simulink library "QD2_Mission_Lib"  (R2022b)
settings: Solver=VariableStepAuto  StartTime=0.0  StopTime=10.0  RelTol=1e-3
undefined symbols (not defined in the file): QD2P
settings Model: Creator=ezequ  LastModifiedBy=ezequ
settings OptimizationCC: ReuseModelBlockBuffer=on
settings RTWCC: GPUComputeCapability=5.0
settings ConfigComp: CovBoundaryAbsTol=1.0e-5

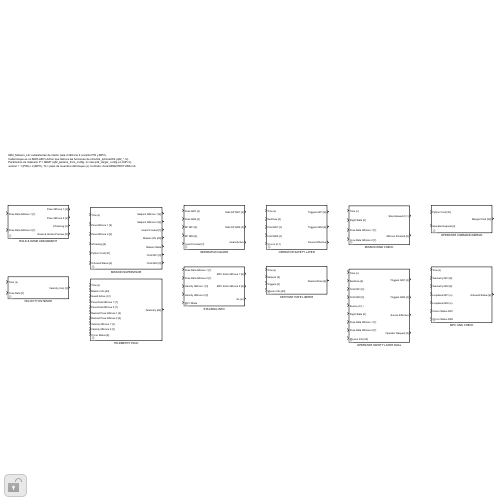
[thumbnail: Simulink's stored preview of the top-level diagram]
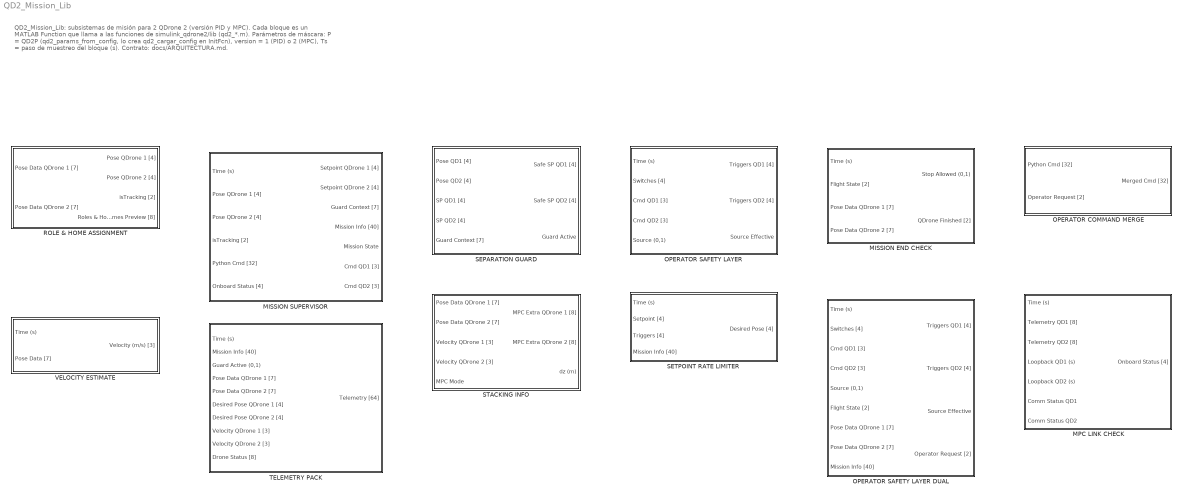
== system QD2_Mission_Lib ==
  note: QD2_Mission_Lib: subsistemas de misión para 2 QDrone 2 (versión PID y MPC).
      | Cada bloque es un MATLAB Function que llama a las funciones de simulink_qdrone2/lib (qd2_*.m).
      | Parámetros de máscara: P = QD2P (qd2_params_from_config, lo crea qd2_cargar_config en InitFcn),
      | version = 1 (PID) o 2 (MPC), Ts = paso de muestreo del bloque (s). Contrato: docs/ARQUITECTURA.md.
  MISSION END CHECK : Subsystem  TreatAsAtomicUnit=on  SystemSampleTime=Ts  mask(QD2 Mission Lib){Ts=0.001}
      mask prompts: Ts "Paso de muestreo (s):"
      mask help: CORRECCIÓN del paro automático del original (paraba 3 s después de Land aunque el dron siguiera en el aire). Un dron "terminó" si su Flight_State es 3 (Land) o 9 (MS Stop) Y está en el suelo (rastreado, z < 0.10 m) durante 3 s seguidos, o lleva 60 s SEGUIDOS sin rastreo en 3/9 (respaldo). Un dron rastreado con z >= 0.10 m NUNCA permite el paro. Stop Allowed = los dos terminaron (o nunca se armaron) y al menos uno se armó. El Stop with Message del Flight Plan solo actúa con Stop Allowed = 1.
  MISSION SUPERVISOR : Subsystem  TreatAsAtomicUnit=on  SystemSampleTime=Ts  mask(QD2 Mission Lib){P=QD2P, version=1, Ts=0.001}
      mask prompts: P "Parámetros de misión (struct de qd2_params_from_config):"; version "Versión (1 = PID, 2 = MPC):"; Ts "Paso de muestreo (s):"
      mask help: FSM de misión (qd2_mission_step, ARQUITECTURA §3.3). Commands = [arm takeoff estop] por dron: el OPERATOR SAFETY LAYER los combina con los switches del operador. Guard Context = [explorer_id ctx_guard(6)]. Onboard Status [4] = [fsm1 fsm2 cod1 cod2] del MPC LINK CHECK (versión MPC; en PID constante 0 = desconocido; cod 1 = protocolo MPC incorrecto, 2 = enlace perdido): un dron en vuelo con FSM a bordo 7/8/9 o sin enlace (o protocolo incorrecto) -> alerta 9 (10), el sano se aparta >= d_min_h a su altura, regresa y aterriza; DONE. En LANDING, R no baja hasta que E está a >= d_min_h en horizontal. Mission Info [40] = campos de telemetría para el TELEMETRY PACK (ver codigo_supervisor en construir_modelos.m).
  MPC LINK CHECK : Subsystem  TreatAsAtomicUnit=on  SystemSampleTime=Ts  mask(QD2 Mission Lib){P=QD2P, version=1, Ts=0.001}
      mask prompts: P "Parámetros de misión (struct de qd2_params_from_config):"; version "Versión (1 = PID, 2 = MPC):"; Ts "Paso de muestreo (s):"
      mask help: Versión MPC (qd2_enlace_mpc): valida la respuesta de 8 doubles de cada dron (§3.2): válida si y(8) = 2 (etiqueta protocolo MPC v1) y la FSM y(2) es un entero 1..9. Si el dron está conectado (loopback < 0.5 s y sin pérdida de enlace) y responde mal más de 0.5 s seguidos -> protocolo incorrecto (cod 1, alerta 10, dron no disponible). Sin conexión después de haber estado conectado -> enlace perdido (cod 2; la FSM retenida no se usa: fsm = 0). Onboard Status = [fsm1 fsm2 cod1 cod2] (fsm 0 = desconocida) -> MISSION SUPERVISOR. Con version = 1 (PID, el dron solo devuelve el eco) la salida es 0.
  OPERATOR COMMAND MERGE : Subsystem  TreatAsAtomicUnit=on  SystemSampleTime=Ts  mask(QD2 Mission Lib){Ts=0.001}
      mask prompts: Ts "Paso de muestreo (s):"
      mask help: Inyecta LAND ALL (cmd 3) en el flujo de comandos de Python cuando el OPERATOR SAFETY LAYER DUAL lo pide (contador Operator Request(1) cambia). Paso 1: heartbeat y cmd_seq distintos -> el supervisor lo acepta aunque la estación Python esté caída. Paso 2: vuelve a la secuencia real de Python SIN comando, así el último comando de Python no se re-ejecuta. La entrada Operator Request debe llegar con 1 paso de retardo.
  OPERATOR SAFETY LAYER : Subsystem  TreatAsAtomicUnit=on  SystemSampleTime=Ts  mask(QD2 Mission Lib){Ts=0.001}
      mask prompts: Ts "Paso de muestreo (s):"
      mask help: Versión SIMPLE (la usa QD2_Sim_Dual; interfaz de 5/3 puertos sin cambios). Los modelos de tierra usan OPERATOR SAFETY LAYER DUAL. En modo MISIÓN (Command Source = 0) arm_i = switch AND misión, takeoff_i = switch AND misión (solo tras >= 1 s armado), estop_i = switch OR misión. En modo MANUAL Equipo2 (1) el dron 1 recibe los switches (takeoff también >= 1 s después de armar) y el dron 2 solo el E-stop. El modo solo cambia con los dos drones desarmados Y los switches Arm y Takeoff abajo (nunca se dispara solo).
  OPERATOR SAFETY LAYER DUAL : Subsystem  TreatAsAtomicUnit=on  SystemSampleTime=Ts  mask(QD2 Mission Lib){P=QD2P, Ts=0.001}
      mask prompts: P "Parámetros de misión (struct de qd2_params_from_config):"; Ts "Paso de muestreo (s):"
      mask help: Capa de seguridad del operador (modelos de tierra). Switches = autoridad final. MISIÓN: arm_i = switch AND misión; Takeoff/Land arriba = PERMISO de despegue (takeoff >= 1 s después de armar); en vuelo, BAJARLO pide LAND ALL al supervisor (Operator Request -> OPERATOR COMMAND MERGE): aterrizaje ordenado, R primero y E se aparta; el takeoff de cada dron sigue al supervisor. Respaldo crudo si el supervisor no acepta en 2 s o tras 90 s: suelta el takeoff, pero NUNCA el de un dron que tiene al otro debajo a < d_min_h. E-stop = corte inmediato. Arm abajo / E-stop en vuelo también piden LAND ALL. MANUAL: como el original (solo dron 1) con takeoff >= 1 s después de armar. El modo solo cambia en tierra: Flight State [0 0], desarmados, switches Arm y Takeoff abajo. Operator Request = [contador de peticiones, alerta 5 E-stop / 6 Takeoff abajo / 7 Arm abajo / 8 respaldo crudo].
  ROLE & HOME ASSIGNMENT : Subsystem  TreatAsAtomicUnit=on  SystemSampleTime=Ts  mask(QD2 Mission Lib){P=QD2P, version=1, Ts=0.001}
      mask prompts: P "Parámetros de misión (struct de qd2_params_from_config):"; version "Versión (1 = PID, 2 = MPC):"; Ts "Paso de muestreo (s):"
      mask help: Separa [x y z yaw] e isTracking de cada dron (Corrected Pose Data [7] = [x y z roll pitch yaw isTracking]) y muestra en vivo la asignación de roles de qd2_assign_roles: [explorer_id responder_id home1(2) home2(2) d_homes start_ok]. El dron con menor x es el EXPLORADOR. El MISSION SUPERVISOR fija roles y homes al recibir START; start_ok = 0 avisa ANTES de START que los homes están demasiado cerca (START se rechazaría, alerta 1).
  SEPARATION GUARD : Subsystem  TreatAsAtomicUnit=on  SystemSampleTime=Ts  mask(QD2 Mission Lib){P=QD2P, Ts=0.001}
      mask prompts: P "Parámetros de misión (struct de qd2_params_from_config):"; Ts "Paso de muestreo (s):"
      mask help: Versión PID: nunca uno encima del otro (qd2_separation_guard). Distancia horizontal >= d_min_h entre poses, consignas y caminos rectos. Traduce dron <-> rol con explorer_id (Guard Context(1)) y reinicia su estado si los roles cambian. Después de este bloque la consigna DEBE limitarse por norma (SETPOINT RATE LIMITER).
  SETPOINT RATE LIMITER : Subsystem  TreatAsAtomicUnit=on  SystemSampleTime=Ts  mask(QD2 Mission Lib){P=QD2P, dron=1, Ts=0.001}
      mask prompts: P "Parámetros de misión (struct de qd2_params_from_config):"; dron "QDrone (1 o 2):"; Ts "Paso de muestreo (s):"
      mask help: Saturation (como Saturation2 original, con z hasta P.z_max) + limitador de razón por NORMA en x,y (qd2_rate_limit(...,1)): 1/3 m/s xy, 1/6 m/s z, 30 °/s yaw. Sustituye al Rate Limiter2 por eje (que hace caminos en L y rompe la separación). Desarmado (Triggers(1) = 0) la consigna pasa sin limitar. Mientras este dron se aparta de un dron en falla a bordo (Mission Info(37 + dron) = 1) el límite xy es P.falla_rate_xy (1 m/s). Parámetro dron = 1 o 2.
  STACKING INFO : Subsystem  TreatAsAtomicUnit=on  SystemSampleTime=Ts  mask(QD2 Mission Lib){Ts=0.001}
      mask prompts: Ts "Paso de muestreo (s):"
      mask help: Versión MPC: índices 17-24 del mensaje de 24 doubles (§3.2) para cada dron = [x y z vx vy vz del OTRO dron, mpc_mode, 2]. El índice 24 = 2 es la etiqueta "protocolo MPC v1": el PROTOCOL CHECK a bordo solo acepta tramas con 24 = 2. Si el otro no está rastreado se mandan NaN (el MPC a bordo desactiva el feedforward de downwash).
  TELEMETRY PACK : Subsystem  TreatAsAtomicUnit=on  SystemSampleTime=Ts  mask(QD2 Mission Lib){version=1, Ts=0.001}
      mask prompts: version "Versión (1 = PID, 2 = MPC):"; Ts "Paso de muestreo (s):"
      mask help: Arma los 64 doubles Simulink -> Python (§3.3) con qd2_telemetry_pack. Drone Status = [fsm1 fsm2 bat1 bat2 comm_issue1 comm_issue2 loopback1 loopback2 (n_peticiones alerta_operador)]; comm_ok = sin issue y loopback < 0.5 s. y(55) = alerta: la del operador (5-8) si hay, si no la del supervisor (0-4, 9 falla a bordo, 10 protocolo MPC incorrecto). y(56:60) = un objetivo por mensaje, rotando: [id clase x y estado]. y(61:63) = [roll pitch válido] del EXPLORADOR (rad), de Pose Data(4:5) del mismo dron (OptiTrack, R = Rz(yaw)Ry(pitch)Rx(roll)); 0 0 0 sin explorador, sin rastreo o con ángulos no finitos. y(64) = 0.
  VELOCITY ESTIMATE : Subsystem  TreatAsAtomicUnit=on  SystemSampleTime=Ts  mask(QD2 Mission Lib){Ts=0.001}
      mask prompts: Ts "Paso de muestreo (s):"
      mask help: Velocidad [vx vy vz] a partir de OptiTrack: derivada entre muestras nuevas (100 Hz) + filtro de primer orden (tau = 0.04 s). Sin rastreo -> 0.

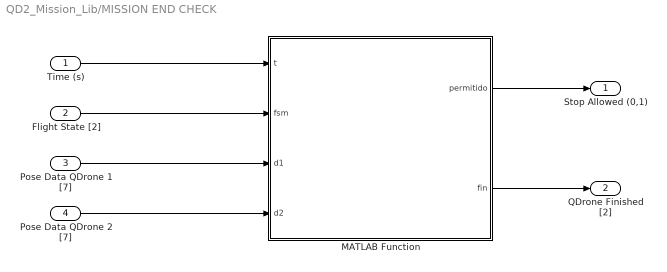
== system QD2_Mission_Lib/MISSION END CHECK ==
  Time (s) : Inport
  Flight State [2] : Inport  Port=2
  Pose Data QDrone 1 [7] : Inport  Port=3
  Pose Data QDrone 2 [7] : Inport  Port=4
  MATLAB Function : MATLAB Function  TreatAsAtomicUnit=on
  Stop Allowed (0,1) : Outport
  QDrone Finished [2] : Outport  Port=2
  wires:
  Time (s)/1 -> MATLAB Function/1(t)
  Flight State [2]/1 -> MATLAB Function/2(fsm)
  Pose Data QDrone 1 [7]/1 -> MATLAB Function/3(d1)
  Pose Data QDrone 2 [7]/1 -> MATLAB Function/4(d2)
  MATLAB Function/1(permitido) -> Stop Allowed (0,1)/1
  MATLAB Function/2(fin) -> QDrone Finished [2]/1

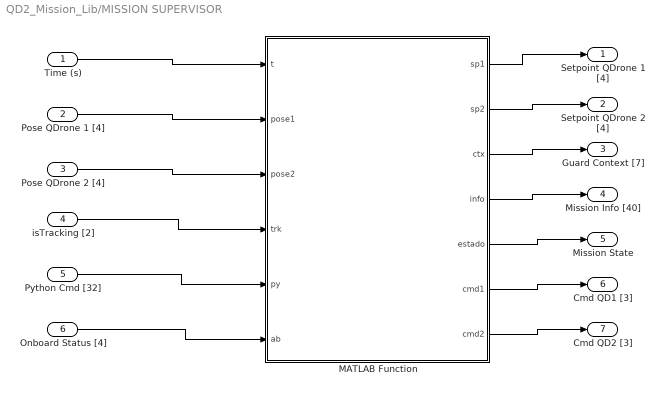
== system QD2_Mission_Lib/MISSION SUPERVISOR ==
  Time (s) : Inport
  Pose QDrone 1 [4] : Inport  Port=2
  Pose QDrone 2 [4] : Inport  Port=3
  isTracking [2] : Inport  Port=4
  Python Cmd [32] : Inport  Port=5
  Onboard Status [4] : Inport  Port=6
  MATLAB Function : MATLAB Function  TreatAsAtomicUnit=on
  Setpoint QDrone 1 [4] : Outport
  Setpoint QDrone 2 [4] : Outport  Port=2
  Guard Context [7] : Outport  Port=3
  Mission Info [40] : Outport  Port=4
  Mission State : Outport  Port=5
  Cmd QD1 [3] : Outport  Port=6
  Cmd QD2 [3] : Outport  Port=7
  wires:
  Time (s)/1 -> MATLAB Function/1(t)
  Pose QDrone 1 [4]/1 -> MATLAB Function/2(pose1)
  Pose QDrone 2 [4]/1 -> MATLAB Function/3(pose2)
  isTracking [2]/1 -> MATLAB Function/4(trk)
  Python Cmd [32]/1 -> MATLAB Function/5(py)
  Onboard Status [4]/1 -> MATLAB Function/6(ab)
  MATLAB Function/1(sp1) -> Setpoint QDrone 1 [4]/1
  MATLAB Function/2(sp2) -> Setpoint QDrone 2 [4]/1
  MATLAB Function/3(ctx) -> Guard Context [7]/1
  MATLAB Function/4(info) -> Mission Info [40]/1
  MATLAB Function/5(estado) -> Mission State/1
  MATLAB Function/6(cmd1) -> Cmd QD1 [3]/1
  MATLAB Function/7(cmd2) -> Cmd QD2 [3]/1

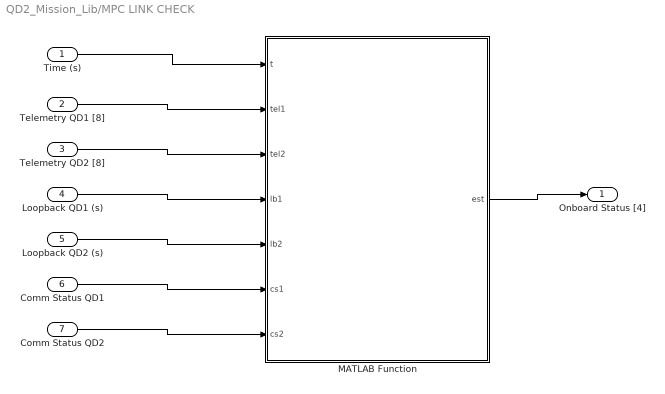
== system QD2_Mission_Lib/MPC LINK CHECK ==
  Time (s) : Inport
  Telemetry QD1 [8] : Inport  Port=2
  Telemetry QD2 [8] : Inport  Port=3
  Loopback QD1 (s) : Inport  Port=4
  Loopback QD2 (s) : Inport  Port=5
  Comm Status QD1 : Inport  Port=6
  Comm Status QD2 : Inport  Port=7
  MATLAB Function : MATLAB Function  TreatAsAtomicUnit=on
  Onboard Status [4] : Outport
  wires:
  Time (s)/1 -> MATLAB Function/1(t)
  Telemetry QD1 [8]/1 -> MATLAB Function/2(tel1)
  Telemetry QD2 [8]/1 -> MATLAB Function/3(tel2)
  Loopback QD1 (s)/1 -> MATLAB Function/4(lb1)
  Loopback QD2 (s)/1 -> MATLAB Function/5(lb2)
  Comm Status QD1/1 -> MATLAB Function/6(cs1)
  Comm Status QD2/1 -> MATLAB Function/7(cs2)
  MATLAB Function/1(est) -> Onboard Status [4]/1

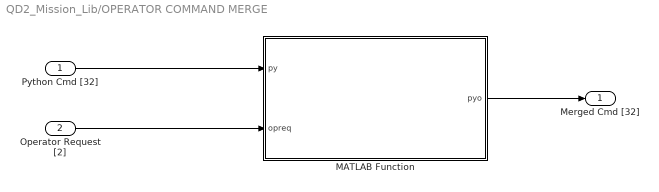
== system QD2_Mission_Lib/OPERATOR COMMAND MERGE ==
  Python Cmd [32] : Inport
  Operator Request [2] : Inport  Port=2
  MATLAB Function : MATLAB Function  TreatAsAtomicUnit=on
  Merged Cmd [32] : Outport
  wires:
  Python Cmd [32]/1 -> MATLAB Function/1(py)
  Operator Request [2]/1 -> MATLAB Function/2(opreq)
  MATLAB Function/1(pyo) -> Merged Cmd [32]/1

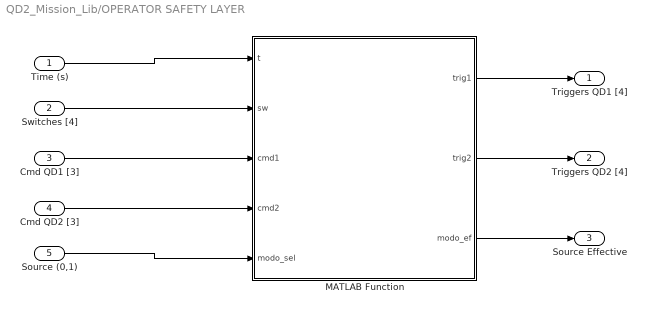
== system QD2_Mission_Lib/OPERATOR SAFETY LAYER ==
  Time (s) : Inport
  Switches [4] : Inport  Port=2
  Cmd QD1 [3] : Inport  Port=3
  Cmd QD2 [3] : Inport  Port=4
  Source (0,1) : Inport  Port=5
  MATLAB Function : MATLAB Function  TreatAsAtomicUnit=on
  Triggers QD1 [4] : Outport
  Triggers QD2 [4] : Outport  Port=2
  Source Effective : Outport  Port=3
  wires:
  Time (s)/1 -> MATLAB Function/1(t)
  Switches [4]/1 -> MATLAB Function/2(sw)
  Cmd QD1 [3]/1 -> MATLAB Function/3(cmd1)
  Cmd QD2 [3]/1 -> MATLAB Function/4(cmd2)
  Source (0,1)/1 -> MATLAB Function/5(modo_sel)
  MATLAB Function/1(trig1) -> Triggers QD1 [4]/1
  MATLAB Function/2(trig2) -> Triggers QD2 [4]/1
  MATLAB Function/3(modo_ef) -> Source Effective/1

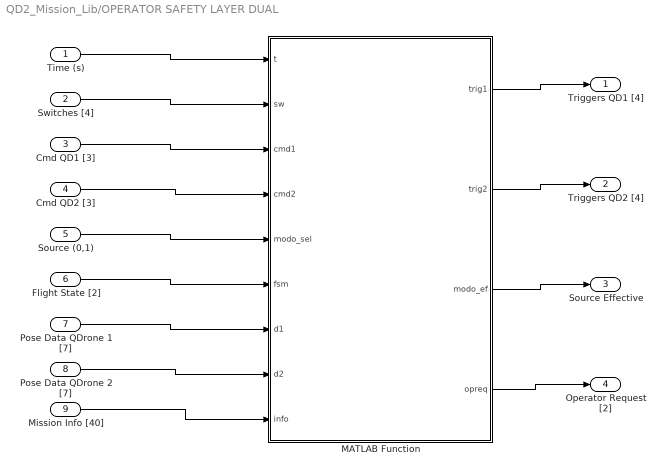
== system QD2_Mission_Lib/OPERATOR SAFETY LAYER DUAL ==
  Time (s) : Inport
  Switches [4] : Inport  Port=2
  Cmd QD1 [3] : Inport  Port=3
  Cmd QD2 [3] : Inport  Port=4
  Source (0,1) : Inport  Port=5
  Flight State [2] : Inport  Port=6
  Pose Data QDrone 1 [7] : Inport  Port=7
  Pose Data QDrone 2 [7] : Inport  Port=8
  Mission Info [40] : Inport  Port=9
  MATLAB Function : MATLAB Function  TreatAsAtomicUnit=on
  Triggers QD1 [4] : Outport
  Triggers QD2 [4] : Outport  Port=2
  Source Effective : Outport  Port=3
  Operator Request [2] : Outport  Port=4
  wires:
  Time (s)/1 -> MATLAB Function/1(t)
  Switches [4]/1 -> MATLAB Function/2(sw)
  Cmd QD1 [3]/1 -> MATLAB Function/3(cmd1)
  Cmd QD2 [3]/1 -> MATLAB Function/4(cmd2)
  Source (0,1)/1 -> MATLAB Function/5(modo_sel)
  Flight State [2]/1 -> MATLAB Function/6(fsm)
  Pose Data QDrone 1 [7]/1 -> MATLAB Function/7(d1)
  Pose Data QDrone 2 [7]/1 -> MATLAB Function/8(d2)
  Mission Info [40]/1 -> MATLAB Function/9(info)
  MATLAB Function/1(trig1) -> Triggers QD1 [4]/1
  MATLAB Function/2(trig2) -> Triggers QD2 [4]/1
  MATLAB Function/3(modo_ef) -> Source Effective/1
  MATLAB Function/4(opreq) -> Operator Request [2]/1

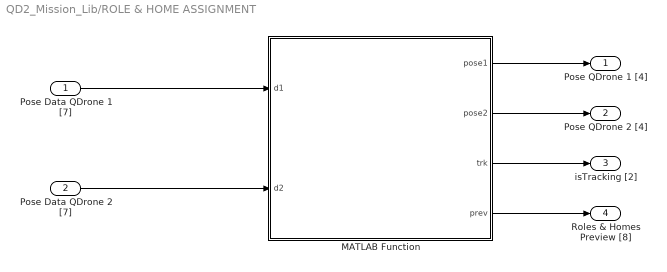
== system QD2_Mission_Lib/ROLE & HOME ASSIGNMENT ==
  Pose Data QDrone 1 [7] : Inport
  Pose Data QDrone 2 [7] : Inport  Port=2
  MATLAB Function : MATLAB Function  TreatAsAtomicUnit=on
  Pose QDrone 1 [4] : Outport
  Pose QDrone 2 [4] : Outport  Port=2
  isTracking [2] : Outport  Port=3
  Roles & Homes Preview [8] : Outport  Port=4
  wires:
  Pose Data QDrone 1 [7]/1 -> MATLAB Function/1(d1)
  Pose Data QDrone 2 [7]/1 -> MATLAB Function/2(d2)
  MATLAB Function/1(pose1) -> Pose QDrone 1 [4]/1
  MATLAB Function/2(pose2) -> Pose QDrone 2 [4]/1
  MATLAB Function/3(trk) -> isTracking [2]/1
  MATLAB Function/4(prev) -> Roles & Homes Preview [8]/1

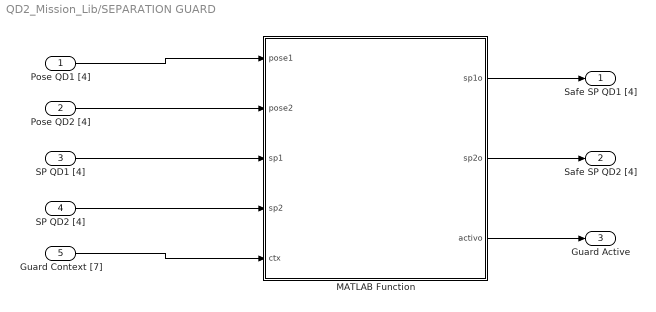
== system QD2_Mission_Lib/SEPARATION GUARD ==
  Pose QD1 [4] : Inport
  Pose QD2 [4] : Inport  Port=2
  SP QD1 [4] : Inport  Port=3
  SP QD2 [4] : Inport  Port=4
  Guard Context [7] : Inport  Port=5
  MATLAB Function : MATLAB Function  TreatAsAtomicUnit=on
  Safe SP QD1 [4] : Outport
  Safe SP QD2 [4] : Outport  Port=2
  Guard Active : Outport  Port=3
  wires:
  Pose QD1 [4]/1 -> MATLAB Function/1(pose1)
  Pose QD2 [4]/1 -> MATLAB Function/2(pose2)
  SP QD1 [4]/1 -> MATLAB Function/3(sp1)
  SP QD2 [4]/1 -> MATLAB Function/4(sp2)
  Guard Context [7]/1 -> MATLAB Function/5(ctx)
  MATLAB Function/1(sp1o) -> Safe SP QD1 [4]/1
  MATLAB Function/2(sp2o) -> Safe SP QD2 [4]/1
  MATLAB Function/3(activo) -> Guard Active/1

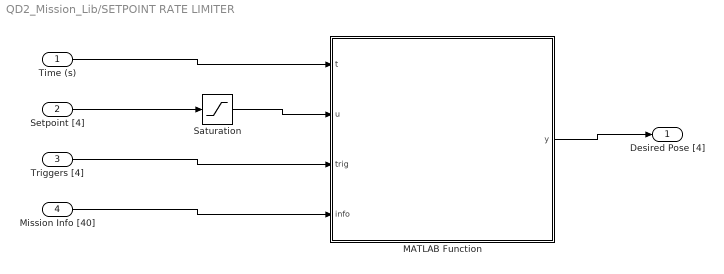
== system QD2_Mission_Lib/SETPOINT RATE LIMITER ==
  Time (s) : Inport
  Setpoint [4] : Inport  Port=2
  Triggers [4] : Inport  Port=3
  Mission Info [40] : Inport  Port=4
  MATLAB Function : MATLAB Function  TreatAsAtomicUnit=on
  Saturation : Saturate  UpperLimit=[P.xy_lim(2); P.xy_lim(2); P.z_max; 3*pi]  LowerLimit=[P.xy_lim(1); P.xy_lim(1); 0; -3*pi]
  Desired Pose [4] : Outport
  wires:
  Time (s)/1 -> MATLAB Function/1(t)
  Setpoint [4]/1 -> Saturation/1
  Saturation/1 -> MATLAB Function/2(u)
  Triggers [4]/1 -> MATLAB Function/3(trig)
  Mission Info [40]/1 -> MATLAB Function/4(info)
  MATLAB Function/1(y) -> Desired Pose [4]/1

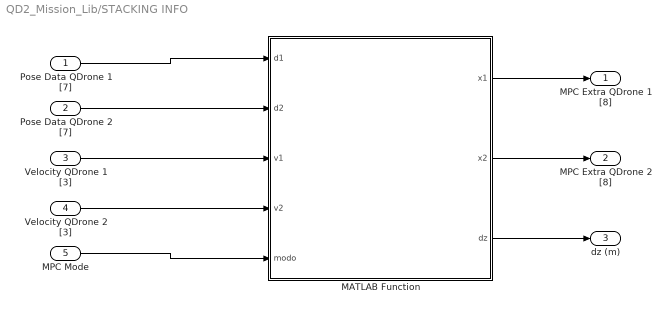
== system QD2_Mission_Lib/STACKING INFO ==
  Pose Data QDrone 1 [7] : Inport
  Pose Data QDrone 2 [7] : Inport  Port=2
  Velocity QDrone 1 [3] : Inport  Port=3
  Velocity QDrone 2 [3] : Inport  Port=4
  MPC Mode : Inport  Port=5
  MATLAB Function : MATLAB Function  TreatAsAtomicUnit=on
  MPC Extra QDrone 1 [8] : Outport
  MPC Extra QDrone 2 [8] : Outport  Port=2
  dz (m) : Outport  Port=3
  wires:
  Pose Data QDrone 1 [7]/1 -> MATLAB Function/1(d1)
  Pose Data QDrone 2 [7]/1 -> MATLAB Function/2(d2)
  Velocity QDrone 1 [3]/1 -> MATLAB Function/3(v1)
  Velocity QDrone 2 [3]/1 -> MATLAB Function/4(v2)
  MPC Mode/1 -> MATLAB Function/5(modo)
  MATLAB Function/1(x1) -> MPC Extra QDrone 1 [8]/1
  MATLAB Function/2(x2) -> MPC Extra QDrone 2 [8]/1
  MATLAB Function/3(dz) -> dz (m)/1

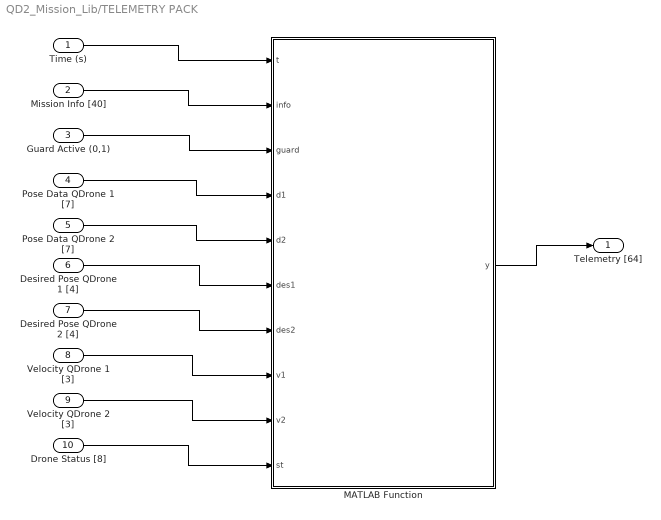
== system QD2_Mission_Lib/TELEMETRY PACK ==
  Time (s) : Inport
  Mission Info [40] : Inport  Port=2
  Guard Active (0,1) : Inport  Port=3
  Pose Data QDrone 1 [7] : Inport  Port=4
  Pose Data QDrone 2 [7] : Inport  Port=5
  Desired Pose QDrone 1 [4] : Inport  Port=6
  Desired Pose QDrone 2 [4] : Inport  Port=7
  Velocity QDrone 1 [3] : Inport  Port=8
  Velocity QDrone 2 [3] : Inport  Port=9
  Drone Status [8] : Inport  Port=10
  MATLAB Function : MATLAB Function  TreatAsAtomicUnit=on
  Telemetry [64] : Outport
  wires:
  Time (s)/1 -> MATLAB Function/1(t)
  Mission Info [40]/1 -> MATLAB Function/2(info)
  Guard Active (0,1)/1 -> MATLAB Function/3(guard)
  Pose Data QDrone 1 [7]/1 -> MATLAB Function/4(d1)
  Pose Data QDrone 2 [7]/1 -> MATLAB Function/5(d2)
  Desired Pose QDrone 1 [4]/1 -> MATLAB Function/6(des1)
  Desired Pose QDrone 2 [4]/1 -> MATLAB Function/7(des2)
  Velocity QDrone 1 [3]/1 -> MATLAB Function/8(v1)
  Velocity QDrone 2 [3]/1 -> MATLAB Function/9(v2)
  Drone Status [8]/1 -> MATLAB Function/10(st)
  MATLAB Function/1(y) -> Telemetry [64]/1

== system QD2_Mission_Lib/VELOCITY ESTIMATE ==
  Time (s) : Inport
  Pose Data [7] : Inport  Port=2
  MATLAB Function : MATLAB Function  TreatAsAtomicUnit=on
  Velocity (m/s) [3] : Outport
  wires:
  Time (s)/1 -> MATLAB Function/1(t)
  Pose Data [7]/1 -> MATLAB Function/2(d)
  MATLAB Function/1(v) -> Velocity (m/s) [3]/1

== matlab function QD2_Mission_Lib/OPERATOR SAFETY LAYER DUAL/MATLAB Function ==
  data: t input; trig1 output size=[1 4]; sw input; cmd1 input; cmd2 input; modo_sel input; fsm input; d1 input; d2 input; info input; trig2 output size=[1 4]; modo_ef output size=1; opreq output size=[2 1]; P parameter
function [trig1, trig2, modo_ef, opreq] = fcn(t, sw, cmd1, cmd2, modo_sel, fsm, d1, d2, info, P)
%#codegen
% OPERATOR SAFETY LAYER DUAL. sw = [Arm Takeoff EStop 0] de los manual switches.
% modo 0 = MISIÓN (2 drones), 1 = MANUAL Equipo2 (solo dron 1, modelo original).
% fsm = Flight State de tierra de cada dron (1 paso de retardo), d1/d2 = Corrected
% Pose Data [x y z roll pitch yaw isTracking], info(1) = estado del MISSION SUPERVISOR.
EXT = true;
D_MIN = P.d_min_h;
estado = info(1);
T_ARM_MIN = 1.0;    % s armado antes de permitir takeoff (a bordo: trigger_2 en IDLE = Error)
T_ACEPTA = 2.0;     % s para que el supervisor acepte el LAND ALL del operador
T_RESPALDO = 90.0;  % s máximos con Takeoff/Land abajo antes del aterrizaje crudo
Z_SUELO = 0.10;     % m
persistent modo t_arm a_prev to_prev sw_prev t_bajo n_req lat_to lat_arm
if isempty(modo)
    modo = double(modo_sel > 0.5);
    t_arm = [-1 -1];
    a_prev = [0 0];
    to_prev = [0 0];
    sw_prev = [double(sw(1) > 0.5) double(sw(2) > 0.5) double(sw(3) > 0.5)];
    t_bajo = -1;
    n_req = 0;
    lat_to = 0;
    lat_arm = 0;
end
sw_arm = sw(1) > 0.5;
sw_to = sw(2) > 0.5;
sw_es = sw(3) > 0.5;
z = [d1(3) d2(3)];
rastreo = [d1(7) > 0.5 && isfinite(d1(3)), d2(7) > 0.5 && isfinite(d2(3))];
armado = a_prev(1) > 0.5 || a_prev(2) > 0.5;
volando = to_prev(1) > 0.5 || to_prev(2) > 0.5;

% ---- Cambio de modo: SOLO en tierra, con los dos Flight State en Idle (0),
% los dos desarmados y los switches Arm y Takeoff ABAJO. Así un cambio del
% selector hecho en vuelo queda pendiente y nunca dispara arm/takeoff solo:
% el operador tiene que bajar los switches y volver a subirlos.
sel = double(modo_sel > 0.5);
suelo = true;
for i = 1:2
    if rastreo(i) && z(i) >= Z_SUELO
        suelo = false;
    end
end
if sel ~= modo && fsm(1) == 0 && fsm(2) == 0 && ~armado && ~volando && ~sw_arm && ~sw_to && suelo
    modo = sel;
    t_arm = [-1 -1];
end

% ---- Peticiones del operador en modo MISIÓN (flancos de los switches)
if EXT && modo < 0.5
    if sw_prev(2) > 0.5 && ~sw_to && (armado || volando)
        n_req = n_req + 1;      % Takeoff/Land abajo -> LAND ALL ordenado
        lat_to = 1;
        t_bajo = t;
    end
    if sw_prev(1) > 0.5 && ~sw_arm && armado
        n_req = n_req + 1;      % Arm abajo (corte, como el original) -> LAND ALL
        lat_arm = 1;
    end
    if sw_prev(3) < 0.5 && sw_es && armado
        n_req = n_req + 1;      % E-stop -> LAND ALL (la misión no sigue)
    end
end
if sw_to
    lat_to = 0;
    t_bajo = -1;
end
if sw_arm
    lat_arm = 0;
end
sw_prev = [double(sw_arm) double(sw_to) double(sw_es)];

% ---- Disparos pedidos
if modo > 0.5
    a = [double(sw_arm) 0];
    to_req = [sw_to false];
    es = [double(sw_es) double(sw_es)];
else
    a = [double(sw_arm && cmd1(1) > 0.5), double(sw_arm && cmd2(1) > 0.5)];
    es = [double(sw_es || cmd1(3) > 0.5), double(sw_es || cmd2(3) > 0.5)];
    if EXT
        % Takeoff/Land = PERMISO para despegar. En vuelo, bajarlo NO corta el
        % takeoff de golpe (cada dron aterrizaría en su x,y: E caería sobre R
        % en la versión MPC); pide LAND ALL y el takeoff sigue al supervisor.
        to_req = [cmd1(2) > 0.5 && (sw_to || to_prev(1) > 0.5), ...
                  cmd2(2) > 0.5 && (sw_to || to_prev(2) > 0.5)];
    else
        to_req = [sw_to && cmd1(2) > 0.5, sw_to && cmd2(2) > 0.5];
    end
end

% ---- Respaldo crudo: el supervisor no aceptó el LAND ALL (estado distinto de
% LANDING/DONE/en tierra) en T_ACEPTA, o pasaron T_RESPALDO con Takeoff abajo.
% Suelta el takeoff, pero NUNCA el de un dron que tiene al otro DEBAJO a
% menos de d_min_h en horizontal (aterrizaría encima / en su downwash).
respaldo = 0;
if EXT && modo < 0.5 && t_bajo >= 0 && volando
    acepto = (estado == 7) || (estado == 8) || (estado <= 2);
    if (~acepto && (t - t_bajo) >= T_ACEPTA) || ((t - t_bajo) >= T_RESPALDO)
        respaldo = 1;
        dh = sqrt((d1(1) - d2(1))^2 + (d1(2) - d2(2))^2);
        for i = 1:2
            o = 3 - i;
            debajo = rastreo(o) && rastreo(i) && dh < D_MIN && z(o) < z(i) - 0.15;
            if ~debajo
                to_req(i) = false;
            end
        end
    end
end

% ---- Takeoff efectivo: >= T_ARM_MIN después de armar (también en MANUAL).
to = [0 0];
for i = 1:2
    if a(i) > 0.5
        if t_arm(i) < 0
            t_arm(i) = t;
        end
    else
        t_arm(i) = -1;
    end
    if modo > 0.5
        % manual: igual que el original una vez en vuelo (el takeoff sigue al
        % switch aunque se baje Arm); para despegar exige 1 s armado
        if to_req(i) && (to_prev(i) > 0.5 || (a(i) > 0.5 && (t - t_arm(i)) >= T_ARM_MIN))
            to(i) = 1;
        end
    elseif to_req(i) && a(i) > 0.5 && (t - t_arm(i)) >= T_ARM_MIN
        to(i) = 1;
    end
end

% ---- Alerta del operador para la telemetría (y(55))
codigo = 0;
if sw_es
    codigo = 5;
elseif respaldo > 0.5
    codigo = 8;
elseif lat_arm > 0.5
    codigo = 7;
elseif lat_to > 0.5
    codigo = 6;
end
a_prev = a;
to_prev = to;
trig1 = [a(1) to(1) es(1) 0];
trig2 = [a(2) to(2) es(2) 0];
modo_ef = modo;
opreq = [n_req; codigo];

== matlab function QD2_Mission_Lib/OPERATOR COMMAND MERGE/MATLAB Function ==
  data: py input; pyo output size=[32 1]; opreq input
function pyo = fcn(py, opreq)
%#codegen
% OPERATOR COMMAND MERGE: inyecta LAND ALL (cmd 3) en los comandos de Python
% cuando el OPERATOR SAFETY LAYER DUAL lo pide (opreq(1) = contador).
persistent n_prev fase
if isempty(n_prev)
    n_prev = opreq(1);
    fase = 0;
end
pyo = zeros(32, 1);
for k = 1:32
    if isfinite(py(k))
        pyo(k) = py(k);
    end
end
if opreq(1) ~= n_prev
    n_prev = opreq(1);
    fase = 1;
end
if fase == 1
    % heartbeat y cmd_seq distintos de los últimos vistos por el supervisor:
    % acepta el LAND ALL aunque la estación Python esté caída
    pyo(1) = pyo(1) + 0.5;
    pyo(2) = 3;
    pyo(3) = pyo(3) + 0.5;
    fase = 2;
elseif fase == 2
    % vuelta a la secuencia real de Python SIN comando: el último comando de
    % Python (p. ej. un START viejo) no se vuelve a ejecutar
    pyo(2) = 0;
    fase = 0;
end

== matlab function QD2_Mission_Lib/SETPOINT RATE LIMITER/MATLAB Function ==
  data: t input; u input; y output size=[1 4]; trig input; info input; P parameter; dron parameter
function y = fcn(t, u, trig, info, P, dron)
%#codegen
% SETPOINT RATE LIMITER: limita x,y por norma (camino recto), z y yaw por eje.
% info(37 + dron) = 1: el dron se aparta de un dron en falla -> límite xy P.falla_rate_xy.
persistent yp tp
uu = [u(1); u(2); u(3); u(4)];
if isempty(yp)
    yp = uu;
    tp = t;
end
dt = t - tp;
if dt < 0
    dt = 0;
end
tp = t;
if ~all(isfinite(uu))
    uu = yp;
end
if trig(1) < 0.5
    yp = uu;   % desarmado: sigue la consigna del supervisor sin limitar
else
    rate = [P.pid.rate_xy; P.pid.rate_xy; P.pid.rate_z; P.pid.rate_yaw];
    ie = min(max(round(37 + dron), 38), 39);
    if info(ie) > 0.5
        rate(1) = P.falla_rate_xy;
        rate(2) = P.falla_rate_xy;
    end
    yp = qd2_rate_limit(yp, uu, rate, dt, 1);
end
% fila [1x4], igual que la salida del Rate Limiter2 original
y = [yp(1) yp(2) yp(3) yp(4)];

== matlab function QD2_Mission_Lib/VELOCITY ESTIMATE/MATLAB Function ==
  data: t input; v output size=[3 1]; d input
function v = fcn(t, d)
%#codegen
% VELOCITY ESTIMATE: derivada entre muestras nuevas de OptiTrack + filtro de 1er orden.
TAU = 0.04;
persistent pl tl vt vf tp
x = [d(1); d(2); d(3)];
if isempty(pl)
    pl = x;
    tl = t - 1;
    vt = zeros(3, 1);
    vf = zeros(3, 1);
    tp = t;
end
dtp = t - tp;
if dtp < 0
    dtp = 0;
end
tp = t;
if all(isfinite(x)) && d(7) > 0.5
    if any(x ~= pl)
        dtm = t - tl;
        if dtm > 1e-4 && dtm < 0.5
            vt = (x - pl)/dtm;
        else
            vt = zeros(3, 1);
        end
        pl = x;
        tl = t;
    elseif t - tl > 0.05
        vt = zeros(3, 1);
    end
else
    vt = zeros(3, 1);
    tl = t - 1;
end
a = dtp/(TAU + dtp);
vf = vf + a*(vt - vf);
v = vf;

== matlab function QD2_Mission_Lib/TELEMETRY PACK/MATLAB Function ==
  data: t input; y output size=[64 1]; info input; guard input; d1 input; d2 input; des1 input; des2 input; v1 input; v2 input; st input; version parameter
function y = fcn(t, info, guard, d1, d2, des1, des2, v1, v2, st, version)
%#codegen
% TELEMETRY PACK: 64 doubles Simulink -> Python (ARQUITECTURA §3.3) con qd2_telemetry_pack.
tel.mission_state = info(1);
tel.explorer_id = info(2);
tel.responder_id = info(3);
tel.explorer_wp_idx = info(4);
tel.explorer_wp_total = info(5);
tel.responder_target_id = info(6);
tel.n_targets_known = info(7);
tel.n_targets_visited = info(8);
tel.explorer_done = info(9);
tel.visited_mask = info(10);
tel.marking_progress = info(11);
tel.queue_length = info(12);
tel.cmd_seq_ack = info(13);
tel.home1 = [info(14) info(15)];
tel.home2 = [info(16) info(17)];
tel.role1 = info(18);
tel.role2 = info(19);
% y(56:60): objetivo de la tabla que toca en este mensaje [id clase x y estado]
tel.obj_rot = [info(33) info(34) info(35) info(36) info(37)];
% alerta: la del operador (Drone Status(10): 5 E-stop, 6 Takeoff abajo, 7 Arm abajo,
% 8 respaldo crudo) tiene prioridad sobre la del supervisor (0-4, 9 falla a bordo,
% 10 protocolo MPC incorrecto)
alerta = info(20);
if numel(st) >= 10
    ov = st(min(10, numel(st)));
    if ov > 0.5
        alerta = ov;
    end
end
tel.alerta = alerta;
pose1 = [d1(1); d1(2); d1(3); d1(6)];
pose2 = [d2(1); d2(2); d2(3); d2(6)];
% comm_ok = sin Communication Issue y loopback < 0.5 s
comm1 = double(st(5) < 0.5 && st(7) < 0.5);
comm2 = double(st(6) < 0.5 && st(8) < 0.5);
aux = [d1(7) d2(7) st(1) st(2) st(3) st(4) comm1 comm2];
% y(61:63): roll y pitch (rad) de la misma Corrected Pose Data [x y z roll pitch yaw trk];
% qd2_telemetry_pack elige los del explorador y pone y(63) = 1 si son válidos
att = [d1(4) d1(5) d2(4) d2(5)];
y = qd2_telemetry_pack(t, tel, version, guard, pose1, pose2, ...
    [des1(1) des1(2) des1(3) des1(4)], [des2(1) des2(2) des2(3) des2(4)], ...
    [v1(1) v1(2) v1(3)], [v2(1) v2(2) v2(3)], aux, att);

== matlab function QD2_Mission_Lib/MISSION END CHECK/MATLAB Function ==
  data: t input; permitido output size=1; fsm input; d1 input; d2 input; fin output size=[2 1]
function [permitido, fin] = fcn(t, fsm, d1, d2)
%#codegen
% MISSION END CHECK: el modelo de tierra solo se detiene con los DOS drones en el suelo.
% Un dron terminó si su Flight_State es 3 (Land) o 9 (MS Stop) y:
%   - está rastreado en el suelo (z < Z_SUELO) T_SUELO s SEGUIDOS, o
%   - lleva T_SIN_RASTREO s SEGUIDOS sin rastreo (respaldo: no se puede confirmar).
% Un dron rastreado con z >= Z_SUELO NUNCA permite el paro (reinicia los dos relojes).
T_SUELO = 3.0;         % s
T_SIN_RASTREO = 60.0;  % s
Z_SUELO = 0.10;        % m
persistent t_suelo t_sin armado
if isempty(armado)
    t_suelo = [-1 -1];
    t_sin = [-1 -1];
    armado = [0 0];
end
z = [d1(3) d2(3)];
trk = [d1(7) d2(7)];
fin = zeros(2, 1);
ok = [false false];
for i = 1:2
    if fsm(i) > 0.5
        armado(i) = 1;
    end
    termino = (fsm(i) == 3) || (fsm(i) == 9);
    rastreado = trk(i) > 0.5 && isfinite(z(i));
    en_suelo = rastreado && z(i) < Z_SUELO;
    if termino && en_suelo
        if t_suelo(i) < 0
            t_suelo(i) = t;
        end
    else
        t_suelo(i) = -1;
    end
    if termino && ~rastreado
        if t_sin(i) < 0
            t_sin(i) = t;
        end
    else
        t_sin(i) = -1;
    end
    fin(i) = double(termino && ((t_suelo(i) >= 0 && (t - t_suelo(i)) >= T_SUELO) || ...
        (t_sin(i) >= 0 && (t - t_sin(i)) >= T_SIN_RASTREO)));
    en_aire = rastreado && z(i) >= Z_SUELO;
    ok(i) = fin(i) > 0.5 || (armado(i) < 0.5 && ~en_aire);
end
permitido = double(ok(1) && ok(2) && (armado(1) > 0.5 || armado(2) > 0.5));

== matlab function QD2_Mission_Lib/MISSION SUPERVISOR/MATLAB Function ==
  data: t input; sp1 output size=[4 1]; pose1 input; pose2 input; trk input; py input; ab input; sp2 output size=[4 1]; ctx output size=[7 1]; info output size=[40 1]; estado output size=1; cmd1 output size=[3 1]; cmd2 output size=[3 1]; P parameter; version parameter
function [sp1, sp2, ctx, info, estado, cmd1, cmd2] = fcn(t, pose1, pose2, trk, py, ab, P, version)
%#codegen
% MISSION SUPERVISOR: qd2_mission_step (FSM de ARQUITECTURA §3.3) para los 2 drones.
% ab = Onboard Status [fsm1 fsm2 cod1 cod2] (MPC LINK CHECK; fsm 0 = desconocida;
% cod 0 bien, 1 protocolo MPC incorrecto, 2 enlace perdido).
persistent s
if isempty(s)
    s = qd2_mission_init(P);
end
in.t = t;
in.pose1 = [pose1(1) pose1(2) pose1(3) pose1(4)];
in.pose2 = [pose2(1) pose2(2) pose2(3) pose2(4)];
in.tracked1 = trk(1);
in.tracked2 = trk(2);
in.py = py(:);
in.version = version;
in.fsm_a_bordo = [ab(1) ab(2)];
in.proto_mal = [ab(3) ab(4)];
[s, ~, ~, tel] = qd2_mission_step(s, in, P);
sp1 = [tel.sp1(1); tel.sp1(2); tel.sp1(3); tel.sp1(4)];
sp2 = [tel.sp2(1); tel.sp2(2); tel.sp2(3); tel.sp2(4)];
cmd1 = [tel.arm(1); tel.takeoff(1); tel.estop(1)];
cmd2 = [tel.arm(2); tel.takeoff(2); tel.estop(2)];
ctx = zeros(7, 1);
ctx(1) = tel.explorer_id;
for k = 1:6
    ctx(k+1) = tel.ctx_guard(k);
end
% Mission Info [40] (orden fijo, lo leen el TELEMETRY PACK, el OPERATOR SAFETY LAYER
% (info(1)) y el SETPOINT RATE LIMITER (info(38:39)))
info = zeros(40, 1);
info(1) = tel.mission_state;      info(2) = tel.explorer_id;
info(3) = tel.responder_id;       info(4) = tel.explorer_wp_idx;
info(5) = tel.explorer_wp_total;  info(6) = tel.responder_target_id;
info(7) = tel.n_targets_known;    info(8) = tel.n_targets_visited;
info(9) = tel.explorer_done;      info(10) = tel.visited_mask;
info(11) = tel.marking_progress;  info(12) = tel.queue_length;
info(13) = tel.cmd_seq_ack;
info(14) = tel.home1(1);  info(15) = tel.home1(2);
info(16) = tel.home2(1);  info(17) = tel.home2(2);
info(18) = tel.role1;     info(19) = tel.role2;
info(20) = tel.alerta;    info(21) = tel.home_ok;
info(22) = tel.pausa_por_trk;  info(23) = tel.hb_ok;
info(24) = tel.pausa_por_hb;   info(25) = tel.z_E;
info(26) = tel.z_R;       info(27) = tel.d_min_h;
info(28) = tel.t_mark;    info(29) = tel.r_marking;
% falla a bordo por dron (0, 9, 10), fase de la reacción, objetivo rotando y(56:60)
info(30) = tel.falla(1);  info(31) = tel.falla(2);
info(32) = tel.falla_fase;
for k = 1:5
    info(32 + k) = tel.obj_rot(k);
end
% 1 = el dron se aparta de un dron en falla (límite xy P.falla_rate_xy)
info(38) = tel.escape(1); info(39) = tel.escape(2);
estado = tel.mission_state;

== matlab function QD2_Mission_Lib/ROLE & HOME ASSIGNMENT/MATLAB Function ==
  data: d1 input; pose1 output size=[4 1]; d2 input; pose2 output size=[4 1]; trk output size=[2 1]; prev output size=[8 1]; P parameter; version parameter
function [pose1, pose2, trk, prev] = fcn(d1, d2, P, version)
%#codegen
% ROLE & HOME ASSIGNMENT. d1/d2 = Corrected Pose Data [x y z roll pitch yaw isTracking].
% prev = [explorer_id responder_id home1x home1y home2x home2y d_homes start_ok] (vista previa;
% el MISSION SUPERVISOR fija roles y homes con START).
pose1 = [d1(1); d1(2); d1(3); d1(6)];
pose2 = [d2(1); d2(2); d2(3); d2(6)];
trk = [d1(7); d2(7)];
[e, r, h1, h2, ok] = qd2_assign_roles(pose1, pose2, trk(1), trk(2));
dh = sqrt((h1(1) - h2(1))^2 + (h1(2) - h2(2))^2);
if version > 1.5
    umbral = P.d_home_min_mpc;
else
    umbral = P.d_min_h + P.guard_margen;
end
prev = [e; r; h1(1); h1(2); h2(1); h2(2); dh; double(ok > 0.5 && dh >= umbral)];

== matlab function QD2_Mission_Lib/SEPARATION GUARD/MATLAB Function ==
  data: pose1 input; sp1o output size=[4 1]; pose2 input; sp1 input; sp2 input; ctx input; sp2o output size=[4 1]; activo output size=1; P parameter
function [sp1o, sp2o, activo] = fcn(pose1, pose2, sp1, sp2, ctx, P)
%#codegen
% SEPARATION GUARD (versión PID): qd2_separation_guard por rol.
persistent gs eid_prev
if isempty(gs)
    gs = qd2_guard_init();
    eid_prev = ctx(1);
end
if ctx(1) ~= eid_prev
    gs = qd2_guard_init();   % los roles cambiaron: el estado ya no aplica
    eid_prev = ctx(1);
end
c6 = [ctx(2) ctx(3) ctx(4) ctx(5) ctx(6) ctx(7)];
p1 = [pose1(1) pose1(2) pose1(3)];
p2 = [pose2(1) pose2(2) pose2(3)];
s1 = [sp1(1) sp1(2) sp1(3) sp1(4)];
s2 = [sp2(1) sp2(2) sp2(3) sp2(4)];
if ctx(1) == 2
    [eO, rO, act, gs] = qd2_separation_guard(p2, p1, s2, s1, P, gs, c6);
    sp1o = [rO(1); rO(2); rO(3); rO(4)];
    sp2o = [eO(1); eO(2); eO(3); eO(4)];
else
    [eO, rO, act, gs] = qd2_separation_guard(p1, p2, s1, s2, P, gs, c6);
    sp1o = [eO(1); eO(2); eO(3); eO(4)];
    sp2o = [rO(1); rO(2); rO(3); rO(4)];
end
activo = double(act);

== matlab function QD2_Mission_Lib/STACKING INFO/MATLAB Function ==
  data: d1 input; x1 output size=[1 8]; d2 input; v1 input; v2 input; modo input; x2 output size=[1 8]; dz output size=1
function [x1, x2, dz] = fcn(d1, d2, v1, v2, modo)
%#codegen
% STACKING INFO (versión MPC): estado del OTRO dron para el MPC a bordo (§3.2, índices 17-24):
% [x y z vx vy vz del otro, mpc_mode, 2].
x1 = zeros(1, 8);
x2 = zeros(1, 8);
if d2(7) > 0.5
    x1(1:3) = [d2(1); d2(2); d2(3)];
    x1(4:6) = [v2(1); v2(2); v2(3)];
else
    x1(1:6) = NaN;
end
if d1(7) > 0.5
    x2(1:3) = [d1(1); d1(2); d1(3)];
    x2(4:6) = [v1(1); v1(2); v1(3)];
else
    x2(1:6) = NaN;
end
x1(7) = modo;
x2(7) = modo;
% índice 24 = 2: etiqueta "protocolo MPC v1" (el PROTOCOL CHECK a bordo solo acepta 2)
x1(8) = 2;
x2(8) = 2;
dz = d1(3) - d2(3);

== matlab function QD2_Mission_Lib/MPC LINK CHECK/MATLAB Function ==
  data: t input; est output size=[4 1]; tel1 input; tel2 input; lb1 input; lb2 input; cs1 input; cs2 input; P parameter; version parameter
function est = fcn(t, tel1, tel2, lb1, lb2, cs1, cs2, P, version)
%#codegen
% MPC LINK CHECK (qd2_enlace_mpc): valida la respuesta de 8 doubles de cada dron
% (§3.2: y(8) = 2, FSM entera 1..9). est = [fsm1 fsm2 cod1 cod2]
% (cod 0 bien, 1 protocolo incorrecto sostenido, 2 enlace perdido).
persistent tm
if isempty(tm)
    tm = [-1 -1 0 0];
end
y1 = zeros(1, 8);
y2 = zeros(1, 8);
for k = 1:8
    y1(k) = tel1(k);
    y2(k) = tel2(k);
end
[e, tm] = qd2_enlace_mpc(tm, t, y1, y2, [lb1(1) lb2(1)], [cs1(1) cs2(1)], P, version);
est = [e(1); e(2); e(3); e(4)];

== matlab function QD2_Mission_Lib/OPERATOR SAFETY LAYER/MATLAB Function ==
  data: t input; trig1 output size=[1 4]; sw input; cmd1 input; cmd2 input; modo_sel input; trig2 output size=[1 4]; modo_ef output size=1
function [trig1, trig2, modo_ef] = fcn(t, sw, cmd1, cmd2, modo_sel)
%#codegen
% OPERATOR SAFETY LAYER (versión simple, interfaz de la simulación QD2_Sim_Dual).
% sw = [Arm Takeoff EStop 0]. modo 0 = MISIÓN, 1 = MANUAL Equipo2 (solo dron 1).
EXT = false;
D_MIN = 0.9;
estado = -1;
fsm = [0 0];
d1 = zeros(7, 1);
d2 = zeros(7, 1);
T_ARM_MIN = 1.0;    % s armado antes de permitir takeoff (a bordo: trigger_2 en IDLE = Error)
T_ACEPTA = 2.0;     % s para que el supervisor acepte el LAND ALL del operador
T_RESPALDO = 90.0;  % s máximos con Takeoff/Land abajo antes del aterrizaje crudo
Z_SUELO = 0.10;     % m
persistent modo t_arm a_prev to_prev sw_prev t_bajo n_req lat_to lat_arm
if isempty(modo)
    modo = double(modo_sel > 0.5);
    t_arm = [-1 -1];
    a_prev = [0 0];
    to_prev = [0 0];
    sw_prev = [double(sw(1) > 0.5) double(sw(2) > 0.5) double(sw(3) > 0.5)];
    t_bajo = -1;
    n_req = 0;
    lat_to = 0;
    lat_arm = 0;
end
sw_arm = sw(1) > 0.5;
sw_to = sw(2) > 0.5;
sw_es = sw(3) > 0.5;
z = [d1(3) d2(3)];
rastreo = [d1(7) > 0.5 && isfinite(d1(3)), d2(7) > 0.5 && isfinite(d2(3))];
armado = a_prev(1) > 0.5 || a_prev(2) > 0.5;
volando = to_prev(1) > 0.5 || to_prev(2) > 0.5;

% ---- Cambio de modo: SOLO en tierra, con los dos Flight State en Idle (0),
% los dos desarmados y los switches Arm y Takeoff ABAJO. Así un cambio del
% selector hecho en vuelo queda pendiente y nunca dispara arm/takeoff solo:
% el operador tiene que bajar los switches y volver a subirlos.
sel = double(modo_sel > 0.5);
suelo = true;
for i = 1:2
    if rastreo(i) && z(i) >= Z_SUELO
        suelo = false;
    end
end
if sel ~= modo && fsm(1) == 0 && fsm(2) == 0 && ~armado && ~volando && ~sw_arm && ~sw_to && suelo
    modo = sel;
    t_arm = [-1 -1];
end

% ---- Peticiones del operador en modo MISIÓN (flancos de los switches)
if EXT && modo < 0.5
    if sw_prev(2) > 0.5 && ~sw_to && (armado || volando)
        n_req = n_req + 1;      % Takeoff/Land abajo -> LAND ALL ordenado
        lat_to = 1;
        t_bajo = t;
    end
    if sw_prev(1) > 0.5 && ~sw_arm && armado
        n_req = n_req + 1;      % Arm abajo (corte, como el original) -> LAND ALL
        lat_arm = 1;
    end
    if sw_prev(3) < 0.5 && sw_es && armado
        n_req = n_req + 1;      % E-stop -> LAND ALL (la misión no sigue)
    end
end
if sw_to
    lat_to = 0;
    t_bajo = -1;
end
if sw_arm
    lat_arm = 0;
end
sw_prev = [double(sw_arm) double(sw_to) double(sw_es)];

% ---- Disparos pedidos
if modo > 0.5
    a = [double(sw_arm) 0];
    to_req = [sw_to false];
    es = [double(sw_es) double(sw_es)];
else
    a = [double(sw_arm && cmd1(1) > 0.5), double(sw_arm && cmd2(1) > 0.5)];
    es = [double(sw_es || cmd1(3) > 0.5), double(sw_es || cmd2(3) > 0.5)];
    if EXT
        % Takeoff/Land = PERMISO para despegar. En vuelo, bajarlo NO corta el
        % takeoff de golpe (cada dron aterrizaría en su x,y: E caería sobre R
        % en la versión MPC); pide LAND ALL y el takeoff sigue al supervisor.
        to_req = [cmd1(2) > 0.5 && (sw_to || to_prev(1) > 0.5), ...
                  cmd2(2) > 0.5 && (sw_to || to_prev(2) > 0.5)];
    else
        to_req = [sw_to && cmd1(2) > 0.5, sw_to && cmd2(2) > 0.5];
    end
end

% ---- Respaldo crudo: el supervisor no aceptó el LAND ALL (estado distinto de
% LANDING/DONE/en tierra) en T_ACEPTA, o pasaron T_RESPALDO con Takeoff abajo.
% Suelta el takeoff, pero NUNCA el de un dron que tiene al otro DEBAJO a
% menos de d_min_h en horizontal (aterrizaría encima / en su downwash).
respaldo = 0;
if EXT && modo < 0.5 && t_bajo >= 0 && volando
    acepto = (estado == 7) || (estado == 8) || (estado <= 2);
    if (~acepto && (t - t_bajo) >= T_ACEPTA) || ((t - t_bajo) >= T_RESPALDO)
        respaldo = 1;
        dh = sqrt((d1(1) - d2(1))^2 + (d1(2) - d2(2))^2);
        for i = 1:2
            o = 3 - i;
            debajo = rastreo(o) && rastreo(i) && dh < D_MIN && z(o) < z(i) - 0.15;
            if ~debajo
                to_req(i) = false;
            end
        end
    end
end

% ---- Takeoff efectivo: >= T_ARM_MIN después de armar (también en MANUAL).
to = [0 0];
for i = 1:2
    if a(i) > 0.5
        if t_arm(i) < 0
            t_arm(i) = t;
        end
    else
        t_arm(i) = -1;
    end
    if modo > 0.5
        % manual: igual que el original una vez en vuelo (el takeoff sigue al
        % switch aunque se baje Arm); para despegar exige 1 s armado
        if to_req(i) && (to_prev(i) > 0.5 || (a(i) > 0.5 && (t - t_arm(i)) >= T_ARM_MIN))
            to(i) = 1;
        end
    elseif to_req(i) && a(i) > 0.5 && (t - t_arm(i)) >= T_ARM_MIN
        to(i) = 1;
    end
end

% ---- Alerta del operador para la telemetría (y(55))
codigo = 0;
if sw_es
    codigo = 5;
elseif respaldo > 0.5
    codigo = 8;
elseif lat_arm > 0.5
    codigo = 7;
elseif lat_to > 0.5
    codigo = 6;
end
a_prev = a;
to_prev = to;
trig1 = [a(1) to(1) es(1) 0];
trig2 = [a(2) to(2) es(2) 0];
modo_ef = modo;
